simulink model "dab_fpga"  (R2024b)
settings: Solver=ode23tb  StartTime=0.0  StopTime=timeSpan  MaxStep=dab_maxstep  RelTol=1e-4
InitFcn:
  | p2s_dir = fileparts(get_param(bdroot, 'FileName'));
  | if ~isempty(p2s_dir), addpath(p2s_dir); end
  | clear p2s_dir
  | dab_params;
values from neighbouring files (symbols this model uses):
  AvergingTime = 1/(SwitchingFrequency/50)    (= 0.000333333333333)    [dab_params.m]
  dab_pid_avg_T = 1/(SwitchingFrequency*0.5)    (= 1.33333333333e-05)    [dab_params.m]
  DeadTime = 100e-9    (= 1e-07)    [dab_params.m]
  Dp = 1.0    (= 1)    [dab_params.m]
  Ds = 0.95    [dab_params.m]
  Force = 1    [dab_params.m]
  n_pri = 11    [dab_params.m]
  n_sec = 4    [dab_params.m]
  Pdab = struct()    [dab_params.m]
  Pout = 16000    [dab_params.m]
  SwitchingFrequency = 150e3    (= 150000)    [dab_params.m]
  tpsDpIntercept = 1.0    (= 1)    [dab_params.m]
  tpsDpMax = 1.0    (= 1)    [dab_params.m]
  tpsDpMin = 1.0    (= 1)    [dab_params.m]
  tpsDpSlope = 0.0    (= 0)    [dab_params.m]
  tpsDsIntercept = 0.95    [dab_params.m]
  tpsDsMax = 0.95    [dab_params.m]
  tpsDsMin = 0.95    [dab_params.m]
  tpsDsSlope = 0.0    (= 0)    [dab_params.m]
  Ts = 1/SwitchingFrequency    (= 6.66666666667e-06)    [dab_params.m]
  Vout = 250    [dab_params.m]
undefined symbols (not defined in the file or in its folder): dab_pid, dab_y0
libraries: slpidlib x1
Description:
  | Ideal-switch translation of DAB FPGA.plecs (see README.md)
settings Model: Creator=Jonathan  LastModifiedBy=Jonathan
settings SolverCC: ZeroCrossAlgorithm=Adaptive
settings DebuggingCC: MaxConsecutiveZCsMsg=none

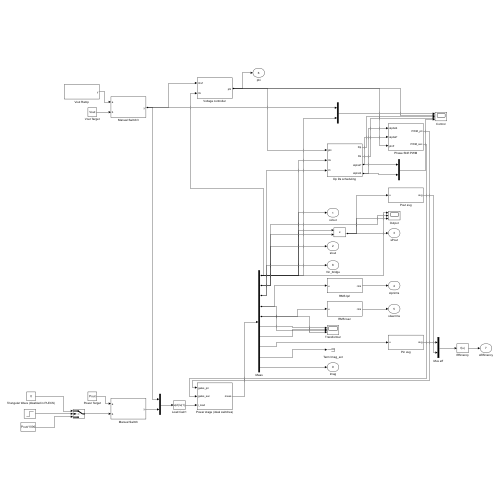
[thumbnail: Simulink's stored preview of the top-level diagram]
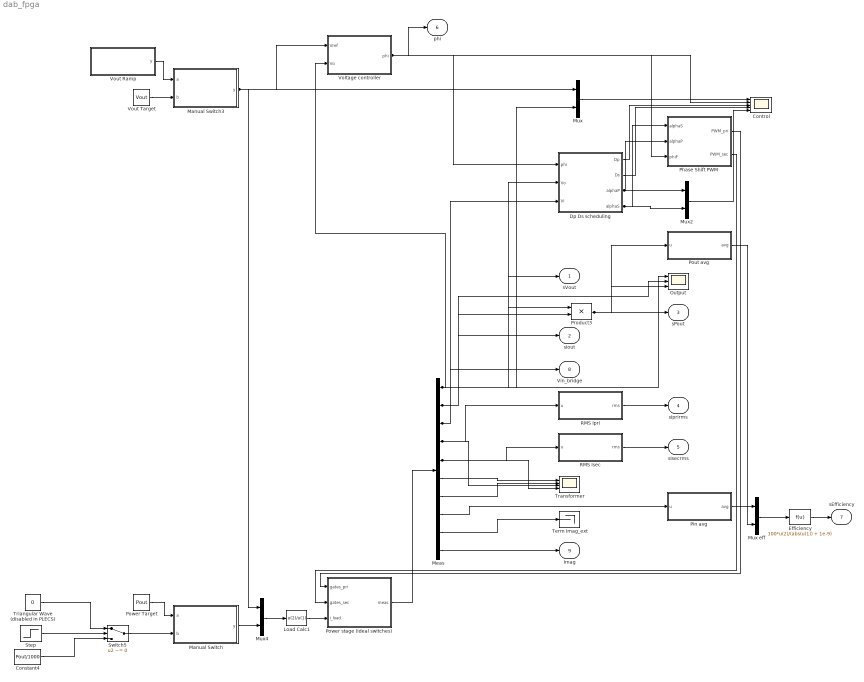
== system dab_fpga ==
  Constant4 : Constant  Value=Pout/1000
  Control : Scope  NumInputPorts=5
  Dp Ds scheduling : Subsystem
  Efficiency : Fcn  Expr=100*u(2)/(abs(u(1)) + 1e-9)
  Load Calc1 : Fcn  Expr=u(2)/u(1)
  Manual Switch : Subsystem
  Manual Switch3 : Subsystem
  Meas : Demux  Outputs=10
  Mux : Mux  Inputs=2
  Mux eff : Mux  Inputs=2
  Mux2 : Mux  Inputs=2
  Mux4 : Mux  Inputs=2
  Output : Scope  NumInputPorts=3
  Phase Shift PWM : Subsystem
  Pin avg : Subsystem
  Pout avg : Subsystem
  Power Target : Constant  Value=Pout
  Power stage (ideal switches) : Subsystem
  Product3 : Product  Inputs=**
  RMS Ipri : Subsystem
  RMS Isec : Subsystem
  Step : Step  Time=0.25  SampleTime=0
  Switch5 : Switch  Criteria=u2 ~= 0  SaturateOnIntegerOverflow=off  InputSameDT=off
  Term Imag_ext : Terminator
  Transformer : Scope  NumInputPorts=4
  Triangular Wave (disabled in PLECS) : Constant  Value=0
  Voltage controller : Subsystem
  Vout Ramp : Subsystem
  Vout Target : Constant  Value=Vout
  sVout : Outport
  sIout : Outport  Port=2
  sPout : Outport  Port=3
  sIprirms : Outport  Port=4
  sIsecrms : Outport  Port=5
  phi : Outport  Port=6
  sEfficiency : Outport  Port=7
  Vin_bridge : Outport  Port=8
  Imag : Outport  Port=9
  wires:
  Switch5/1 -> Manual Switch/2(b)
  Constant4/1 -> Switch5/3
  Power Target/1 -> Manual Switch/1(a)
  Step/1 -> Switch5/2
  Triangular Wave (disabled in PLECS)/1 -> Switch5/1
  Meas/7 -> Transformer/2
  Vout Ramp/1(y) -> Manual Switch3/1(a)
  Manual Switch3/1(y) -> Mux/1, Mux4/1, Voltage controller/1(Vref)
  Mux/1 -> Control/1
  Vout Target/1 -> Manual Switch3/2(b)
  RMS Ipri/1(rms) -> sIprirms/1
  Load Calc1/1 -> Power stage (ideal switches)/3(i_load)
  Manual Switch/1(y) -> Mux4/2
  Mux4/1 -> Load Calc1/1
  Voltage controller/1(phi) -> Control/2, Phase Shift PWM/3(phiF), Dp Ds scheduling/1(phi), phi/1
  Power stage (ideal switches)/1(meas) -> Meas/1
  Efficiency/1 -> sEfficiency/1
  Dp Ds scheduling/2(Ds) -> Control/4
  Meas/1 -> Voltage controller/2(Vo), Dp Ds scheduling/2(Vo), Product3/1, Output/1, sVout/1, Mux/2
  Meas/10 -> Imag/1
  Meas/2 -> Output/2, Product3/2, sIout/1
  Mux eff/1 -> Efficiency/1
  Meas/3 -> Vin_bridge/1, Dp Ds scheduling/3(Vi)
  Meas/4 -> RMS Ipri/1(u), Transformer/3
  Meas/5 -> RMS Isec/1(u), Transformer/4
  Mux2/1 -> Control/5
  Meas/6 -> Transformer/1
  Dp Ds scheduling/3(alphaP) -> Phase Shift PWM/2(alphaP), Mux2/1
  Meas/8 -> Pin avg/1(u)
  Product3/1 -> Pout avg/1(u), Output/3, sPout/1
  Meas/9 -> Term Imag_ext/1
  Dp Ds scheduling/1(Dp) -> Control/3
  Dp Ds scheduling/4(alphaS) -> Phase Shift PWM/1(alphaS), Mux2/2
  RMS Isec/1(rms) -> sIsecrms/1
  Phase Shift PWM/1(PWM_pri) -> Power stage (ideal switches)/1(gates_pri)
  Phase Shift PWM/2(PWM_sec) -> Power stage (ideal switches)/2(gates_sec)
  Pout avg/1(avg) -> Mux eff/2
  Pin avg/1(avg) -> Mux eff/1

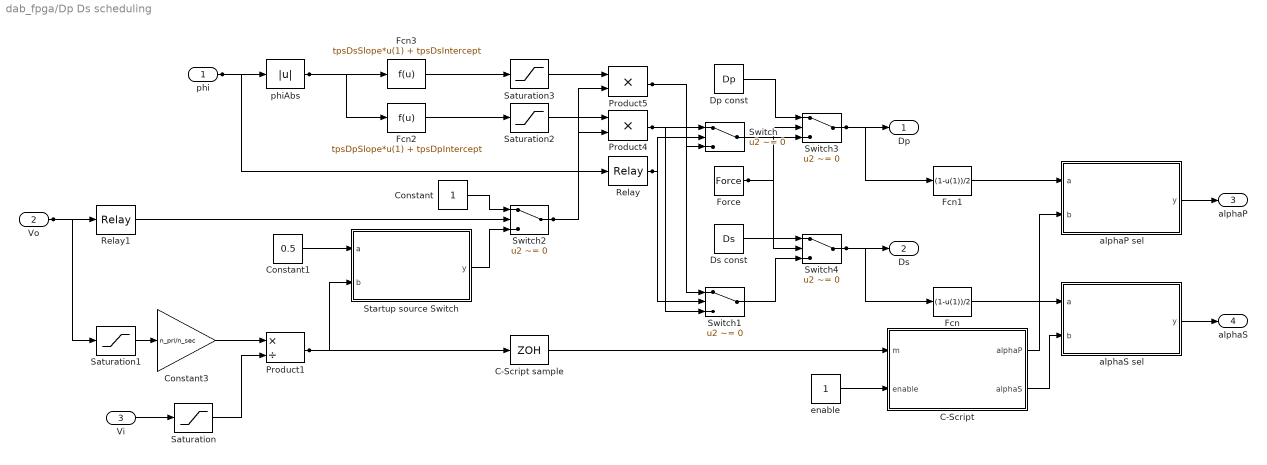
== system dab_fpga/Dp Ds scheduling ==
  phi : Inport
  Vo : Inport  Port=2
  Vi : Inport  Port=3
  C-Script : MATLAB Function  TreatAsAtomicUnit=on
  C-Script sample : ZeroOrderHold  SampleTime=Ts/10
  Constant : Constant
  Constant1 : Constant  Value=0.5
  Constant3 : Gain  Gain=n_pri/n_sec
  Dp const : Constant  Value=Dp
  Ds const : Constant  Value=Ds
  Fcn : Fcn  Expr=(1-u(1))/2
  Fcn1 : Fcn  Expr=(1-u(1))/2
  Fcn2 : Fcn  Expr=tpsDpSlope*u(1) + tpsDpIntercept
  Fcn3 : Fcn  Expr=tpsDsSlope*u(1) + tpsDsIntercept
  Force : Constant  Value=Force
  Product1 : Product  Inputs=*/
  Product4 : Product  Inputs=**
  Product5 : Product  Inputs=**
  Relay : Relay  OnSwitchValue=0.01  OffSwitchValue=-0.01
  Relay1 : Relay  OnSwitchValue=Vout  OffSwitchValue=Vout - 150
  Saturation : Saturate  UpperLimit=inf  LowerLimit=1
  Saturation1 : Saturate  UpperLimit=inf  LowerLimit=50
  Saturation2 : Saturate  UpperLimit=tpsDpMax  LowerLimit=tpsDpMin
  Saturation3 : Saturate  UpperLimit=tpsDsMax  LowerLimit=tpsDsMin
  Startup source Switch : Subsystem
  Switch{,1..4} (5 alike) : Switch  Criteria=u2 ~= 0  SaturateOnIntegerOverflow=off  InputSameDT=off
  alphaP sel : Subsystem
  alphaS sel : Subsystem
  enable : Constant
  phiAbs : Abs  SaturateOnIntegerOverflow=off
  Dp : Outport
  Ds : Outport  Port=2
  alphaP : Outport  Port=3
  alphaS : Outport  Port=4
  wires:
  Vo/1 -> Relay1/1, Saturation1/1
  Saturation1/1 -> Constant3/1
  Relay1/1 -> Switch2/2
  Vi/1 -> Saturation/1
  Saturation/1 -> Product1/2
  phi/1 -> Relay/1, phiAbs/1
  phiAbs/1 -> Fcn2/1, Fcn3/1
  Constant3/1 -> Product1/1
  Constant1/1 -> Startup source Switch/1(a)
  Product1/1 -> C-Script sample/1, Startup source Switch/2(b)
  Fcn3/1 -> Saturation3/1
  Fcn2/1 -> Saturation2/1
  Constant/1 -> Switch2/1
  Startup source Switch/1(y) -> Switch2/3
  Relay/1 -> Switch/2, Switch1/2
  Saturation3/1 -> Product5/1
  Saturation2/1 -> Product4/1
  Switch2/1 -> Product4/2, Product5/2
  C-Script sample/1 -> C-Script/1(m)
  Force/1 -> Switch3/2, Switch4/2
  Product5/1 -> Switch/3, Switch1/1
  Product4/1 -> Switch/1, Switch1/3
  Dp const/1 -> Switch3/1
  Switch/1 -> Switch3/3
  Ds const/1 -> Switch4/1
  Switch1/1 -> Switch4/3
  Switch3/1 -> Fcn1/1, Dp/1
  Switch4/1 -> Ds/1, Fcn/1
  enable/1 -> C-Script/2(enable)
  Fcn1/1 -> alphaP sel/1(a)
  Fcn/1 -> alphaS sel/1(a)
  C-Script/1(alphaP) -> alphaP sel/2(b)
  C-Script/2(alphaS) -> alphaS sel/2(b)
  alphaP sel/1(y) -> alphaP/1
  alphaS sel/1(y) -> alphaS/1

== system dab_fpga/Manual Switch ==
  a : Inport
  b : Inport  Port=2
  Switch : Switch  Criteria=u2 > Threshold  Threshold=0.5  SaturateOnIntegerOverflow=off  InputSameDT=off
  sel : Constant  Value=double(sel_power == 1)
  y : Outport
  wires:
  b/1 -> Switch/3
  a/1 -> Switch/1
  Switch/1 -> y/1
  sel/1 -> Switch/2

== system dab_fpga/Manual Switch3 ==
  a : Inport
  b : Inport  Port=2
  Switch : Switch  Criteria=u2 > Threshold  Threshold=0.5  SaturateOnIntegerOverflow=off  InputSameDT=off
  sel : Constant  Value=double(sel_vref == 1)
  y : Outport
  wires:
  Switch/1 -> y/1
  b/1 -> Switch/3
  sel/1 -> Switch/2
  a/1 -> Switch/1

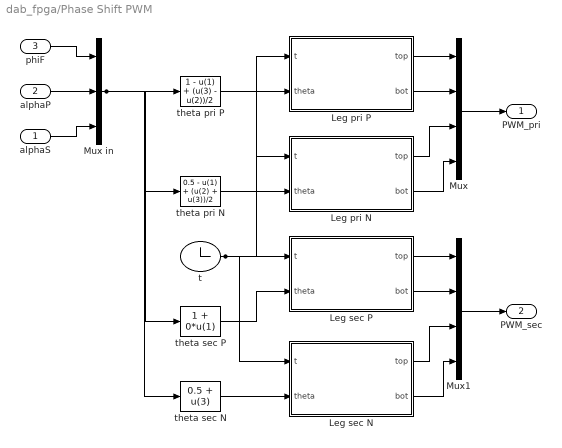
== system dab_fpga/Phase Shift PWM ==
  alphaS : Inport
  alphaP : Inport  Port=2
  phiF : Inport  Port=3
  Leg pri N : Subsystem
  Leg pri P : Subsystem
  Leg sec N : Subsystem
  Leg sec P : Subsystem
  Mux : Mux
  Mux in : Mux  Inputs=3
  Mux1 : Mux
  t : Clock
  theta pri N : Fcn  Expr=0.5 - u(1) + (u(2) + u(3))/2
  theta pri P : Fcn  Expr=1 - u(1) + (u(3) - u(2))/2
  theta sec N : Fcn  Expr=0.5 + u(3)
  theta sec P : Fcn  Expr=1 + 0*u(1)
  PWM_pri : Outport
  PWM_sec : Outport  Port=2
  wires:
  phiF/1 -> Mux in/1
  theta pri N/1 -> Leg pri N/2(theta)
  alphaP/1 -> Mux in/2
  theta sec P/1 -> Leg sec P/2(theta)
  alphaS/1 -> Mux in/3
  Mux in/1 -> theta pri P/1, theta pri N/1, theta sec P/1, theta sec N/1
  theta pri P/1 -> Leg pri P/2(theta)
  t/1 -> Leg pri P/1(t), Leg sec P/1(t), Leg pri N/1(t), Leg sec N/1(t)
  theta sec N/1 -> Leg sec N/2(theta)
  Leg pri P/1(top) -> Mux/1
  Leg pri P/2(bot) -> Mux/2
  Leg pri N/1(top) -> Mux/3
  Leg pri N/2(bot) -> Mux/4
  Leg sec P/1(top) -> Mux1/1
  Leg sec P/2(bot) -> Mux1/2
  Leg sec N/1(top) -> Mux1/3
  Leg sec N/2(bot) -> Mux1/4
  Mux/1 -> PWM_pri/1
  Mux1/1 -> PWM_sec/1

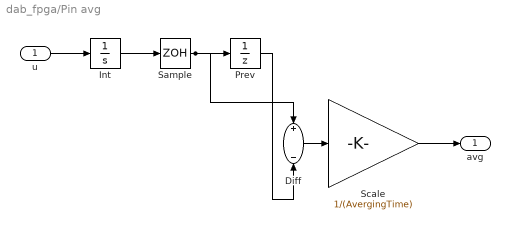
== system dab_fpga/Pin avg ==
  u : Inport
  Diff : Sum  Inputs=+-
  Int : Integrator
  Prev : UnitDelay  SampleTime=AvergingTime  HasFrameUpgradeWarning=on
  Sample : ZeroOrderHold  SampleTime=AvergingTime
  Scale : Gain  Gain=1/(AvergingTime)
  avg : Outport
  wires:
  u/1 -> Int/1
  Int/1 -> Sample/1
  Sample/1 -> Diff/1, Prev/1
  Prev/1 -> Diff/2
  Diff/1 -> Scale/1
  Scale/1 -> avg/1

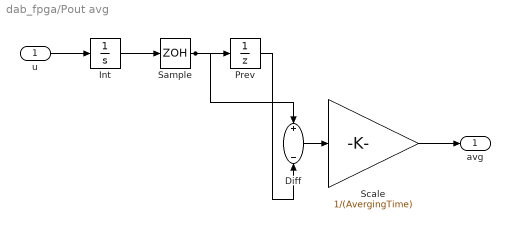
== system dab_fpga/Pout avg ==
  u : Inport
  Diff : Sum  Inputs=+-
  Int : Integrator
  Prev : UnitDelay  SampleTime=AvergingTime  HasFrameUpgradeWarning=on
  Sample : ZeroOrderHold  SampleTime=AvergingTime
  Scale : Gain  Gain=1/(AvergingTime)
  avg : Outport
  wires:
  Diff/1 -> Scale/1
  u/1 -> Int/1
  Int/1 -> Sample/1
  Sample/1 -> Diff/1, Prev/1
  Prev/1 -> Diff/2
  Scale/1 -> avg/1

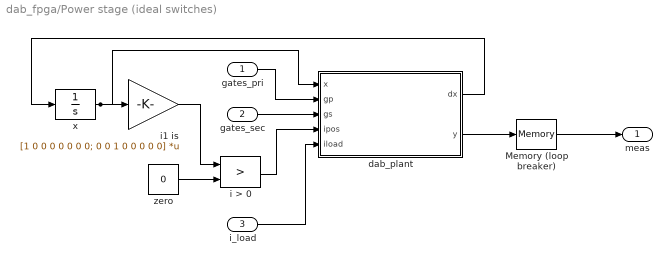
== system dab_fpga/Power stage (ideal switches) ==
  gates_pri : Inport
  gates_sec : Inport  Port=2
  i_load : Inport  Port=3
  Memory (loop breaker) : Memory  InitialCondition=dab_y0
  dab_plant : MATLAB Function  TreatAsAtomicUnit=on
  i > 0 : RelationalOperator  Operator=>  OutDataTypeStr=boolean  RndMeth=Simplest  InputSameDT=off
  i1 is : Gain  Gain=[1 0 0 0 0 0 0 0; 0 0 1 0 0 0 0 0]  Multiplication=Matrix(K*u)
  x : Integrator  InitialCondition=Pdab.x0
  zero : Constant  Value=0
  meas : Outport
  wires:
  i1 is/1 -> i > 0/1
  x/1 -> dab_plant/1(x), i1 is/1
  zero/1 -> i > 0/2
  gates_sec/1 -> dab_plant/3(gs)
  gates_pri/1 -> dab_plant/2(gp)
  i > 0/1 -> dab_plant/4(ipos)
  i_load/1 -> dab_plant/5(iload)
  dab_plant/1(dx) -> x/1
  dab_plant/2(y) -> Memory (loop breaker)/1
  Memory (loop breaker)/1 -> meas/1

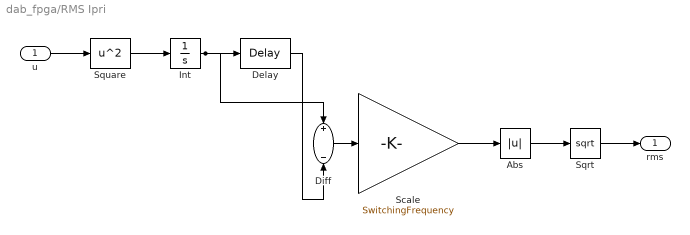
== system dab_fpga/RMS Ipri ==
  u : Inport
  Abs : Abs  SaturateOnIntegerOverflow=off
  Delay : TransportDelay  DelayTime=1/(SwitchingFrequency)  BufferSize=131072
  Diff : Sum  Inputs=+-
  Int : Integrator
  Scale : Gain  Gain=SwitchingFrequency
  Sqrt : Sqrt
  Square : Math  Operator=square
  rms : Outport
  wires:
  u/1 -> Square/1
  Scale/1 -> Abs/1
  Square/1 -> Int/1
  Abs/1 -> Sqrt/1
  Int/1 -> Diff/1, Delay/1
  Sqrt/1 -> rms/1
  Delay/1 -> Diff/2
  Diff/1 -> Scale/1

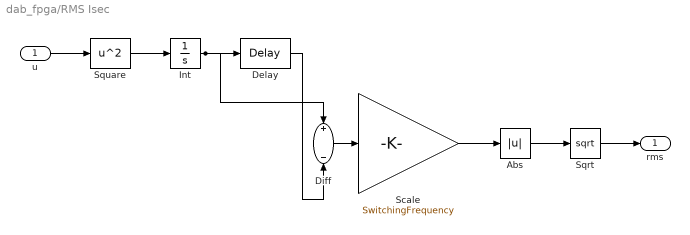
== system dab_fpga/RMS Isec ==
  u : Inport
  Abs : Abs  SaturateOnIntegerOverflow=off
  Delay : TransportDelay  DelayTime=1/(SwitchingFrequency)  BufferSize=131072
  Diff : Sum  Inputs=+-
  Int : Integrator
  Scale : Gain  Gain=SwitchingFrequency
  Sqrt : Sqrt
  Square : Math  Operator=square
  rms : Outport
  wires:
  Diff/1 -> Scale/1
  u/1 -> Square/1
  Abs/1 -> Sqrt/1
  Square/1 -> Int/1
  Sqrt/1 -> rms/1
  Int/1 -> Diff/1, Delay/1
  Delay/1 -> Diff/2
  Scale/1 -> Abs/1

== system dab_fpga/Voltage controller ==
  Vref : Inport
  Vo : Inport  Port=2
  Continuous PID Controller : slpidlib/PID Controller  Controller=PI  Form=Parallel  TimeDomain=Continuous-time  UseExternalTs=off  SampleTime=-1  IntegratorMethod=Forward Euler  FilterMethod=Forward Euler  ControllerParametersSource=internal  P=dab_pid.kp  I=dab_pid.ki  UseKiTs=off  D=0  UseExternalDerivativeSource=off  N=100  UseFilter=on  TunerSelectOption=Transfer Function Based (PID Tuner App)  InitialConditionSource=internal  InitialConditionForIntegrator=dab_pid.x0  InitialConditionForFilter=0  DifferentiatorICPrevScaledInput=0  ExternalReset=none  TrackingMode=off  Kt=1  LimitOutput=on  SatLimitsSource=internal  UpperSaturationLimit=dab_pid.up  LowerSaturationLimit=dab_pid.lo  LinearizeAsGain=on  AntiWindupMode=back-calculation  Kb=dab_pid.kbc  LimitIntegrator=off  UpperIntegratorSaturationLimit=inf  LowerIntegratorSaturationLimit=-inf  POutMin=[]  POutMax=[]  IOutMin=[]  IOutMax=[]  DOutMin=[]  DOutMax=[]  NOutMin=[]  NOutMax=[]  SumOutMin=[]  SumOutMax=[]  SaturationOutMin=[]  SaturationOutMax=[]  PParamMin=[]  PParamMax=[]  IParamMin=[]  IParamMax=[]  DParamMin=[]  DParamMax=[]  NParamMin=[]  NParamMax=[]  KbParamMin=[]  KbParamMax=[]  KtParamMin=[]  KtParamMax=[]  KbOutMin=[]  KbOutMax=[]  KtOutMin=[]  KtOutMax=[]  IntegratorOutMin=[]  IntegratorOutMax=[]  FilterOutMin=[]  FilterOutMax=[]  SumI1OutMin=[]  SumI1OutMax=[]  SumI2OutMin=[]  SumI2OutMax=[]  SumI3OutMin=[]  SumI3OutMax=[]  SumI4OutMin=[]  SumI4OutMax=[]  SumDOutMin=[]  SumDOutMax=[]  DifferentiatorOutMin=[]  DifferentiatorOutMax=[]  FilterDiffOutCoefMin=[]  FilterDiffOutCoefMax=[]  ReciprocalOutMin=[]  ReciprocalOutMax=[]  SumDenOutMin=[]  SumDenOutMax=[]  SumNumOutMin=[]  SumNumOutMax=[]  DivideOutMin=[]  DivideOutMax=[]  UdiffTsProdOutMin=[]  UdiffTsProdOutMax=[]  NTsProdOutMin=[]  NTsProdOutMax=[]  UintegralTsProdOutMin=[]  UintegralTsProdOutMax=[]  UngainTsProdOutMin=[]  UngainTsProdOutMax=[]  ClampingZeroOutDataTypeStr=Inherit: Inherit via back propagation  ClampingZeroOutMin=[]  ClampingZeroOutMax=[]  FilterDenConstantOutDataTypeStr=Inherit: Inherit via back propagation  FilterDenConstantOutMin=[]  FilterDenConstantOutMax=[]  PCopyOutDataTypeStr=Inherit: Inherit via back propagation  PCopyOutMin=[]  PCopyOutMax=[]  NCopyOutDataTypeStr=Inherit: Inherit via back propagation  NCopyOutMin=[]  NCopyOutMax=[]  IntegratorContinuousStateAttributes=''  IntegratorStateMustResolveToSignalObject=off  IntegratorRTWStateStorageClass=Auto  FilterContinuousStateAttributes=''  FilterStateMustResolveToSignalObject=off  FilterRTWStateStorageClass=Auto  ParallelPVariant=InternalParameters  IdealPVariant=Disabled  IVariant=InternalParameters  DVariant=Disabled  IntegratorVariant=Continuous  SatVariant=Enabled  AWVariant=BackCalculation  PCopyVariant=Disabled  TRVariant=Disabled  FdbkBlocksVariant=Forward  IdealPFdbkVariant=Disabled  SatFdbkVariant=Disabled  DerivativeFilterVariant=Disabled  NVariant=Disabled  NCopyVariant=Disabled_SignalSpec  FilterICVariant=Disabled  IntegratorICVariant=InternalICs  ExternalResetVariant=Disabled  TRSumVariant=Passthrough  SumFdbkVariant=Disabled  SumVariant=Sum_PI  TsampFilterVariant=InternalTs  TsampNgainVariant=Passthrough  TsampIntegralVariant=Disabled_SignalSpec  ExternalSaturationOutDataTypeStr=Inherit: Same as second input  DerivativeSourceVariant=Disabled  PreIntVariant=InternalPreInt
  Gain : Gain  Gain=0.5
  Periodic Average5 : Subsystem
  Sum2 : Sum  Inputs=+-
  phi : Outport
  wires:
  Vref/1 -> Sum2/1
  Gain/1 -> phi/1
  Periodic Average5/1(avg) -> Continuous PID Controller/1
  Sum2/1 -> Periodic Average5/1(u)
  Vo/1 -> Sum2/2
  Continuous PID Controller/1 -> Gain/1

== system dab_fpga/Vout Ramp ==
  Limit : Saturate  UpperLimit=max(0.1,Vout)  LowerLimit=min(0.1,Vout)
  Ramp : Fcn  Expr=(0.1) + (1600)*(u(1)-(0.0))*(u(1)>(0.0))
  t : Clock
  y : Outport
  wires:
  t/1 -> Ramp/1
  Ramp/1 -> Limit/1
  Limit/1 -> y/1

== system dab_fpga/Dp Ds scheduling/Startup source Switch ==
  a : Inport
  b : Inport  Port=2
  Switch : Switch  Criteria=u2 > Threshold  Threshold=0.5  SaturateOnIntegerOverflow=off  InputSameDT=off
  sel : Constant  Value=double(sel_startup == 1)
  y : Outport
  wires:
  a/1 -> Switch/1
  sel/1 -> Switch/2
  b/1 -> Switch/3
  Switch/1 -> y/1

== system dab_fpga/Dp Ds scheduling/alphaP sel ==
  a : Inport
  b : Inport  Port=2
  Switch : Switch  Criteria=u2 > Threshold  Threshold=0.5  SaturateOnIntegerOverflow=off  InputSameDT=off
  sel : Constant  Value=double(sel_alphaP == 1)
  y : Outport
  wires:
  a/1 -> Switch/1
  sel/1 -> Switch/2
  b/1 -> Switch/3
  Switch/1 -> y/1

== system dab_fpga/Dp Ds scheduling/alphaS sel ==
  a : Inport
  b : Inport  Port=2
  Switch : Switch  Criteria=u2 > Threshold  Threshold=0.5  SaturateOnIntegerOverflow=off  InputSameDT=off
  sel : Constant  Value=double(sel_alphaS == 1)
  y : Outport
  wires:
  a/1 -> Switch/1
  Switch/1 -> y/1
  sel/1 -> Switch/2
  b/1 -> Switch/3

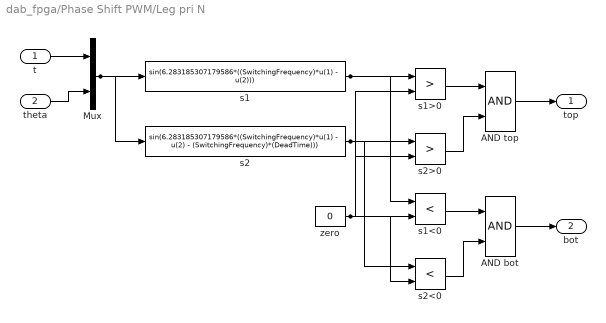
== system dab_fpga/Phase Shift PWM/Leg pri N ==
  t : Inport
  theta : Inport  Port=2
  AND bot : Logic  AllPortsSameDT=off  OutDataTypeStr=boolean
  AND top : Logic  AllPortsSameDT=off  OutDataTypeStr=boolean
  Mux : Mux  Inputs=2
  s1 : Fcn  Expr=sin(6.283185307179586*((SwitchingFrequency)*u(1) - u(2)))
  s1<0 : RelationalOperator  Operator=<  OutDataTypeStr=boolean  RndMeth=Simplest  InputSameDT=off
  s1>0 : RelationalOperator  Operator=>  OutDataTypeStr=boolean  RndMeth=Simplest  InputSameDT=off
  s2 : Fcn  Expr=sin(6.283185307179586*((SwitchingFrequency)*u(1) - u(2) - (SwitchingFrequency)*(DeadTime)))
  s2<0 : RelationalOperator  Operator=<  OutDataTypeStr=boolean  RndMeth=Simplest  InputSameDT=off
  s2>0 : RelationalOperator  Operator=>  OutDataTypeStr=boolean  RndMeth=Simplest  InputSameDT=off
  zero : Constant  Value=0
  top : Outport
  bot : Outport  Port=2
  wires:
  t/1 -> Mux/1
  theta/1 -> Mux/2
  s2>0/1 -> AND top/2
  zero/1 -> s2>0/2, s1>0/2, s1<0/2, s2<0/2
  Mux/1 -> s1/1, s2/1
  s1/1 -> s1>0/1, s1<0/1
  s2/1 -> s2>0/1, s2<0/1
  s1>0/1 -> AND top/1
  s1<0/1 -> AND bot/1
  s2<0/1 -> AND bot/2
  AND top/1 -> top/1
  AND bot/1 -> bot/1

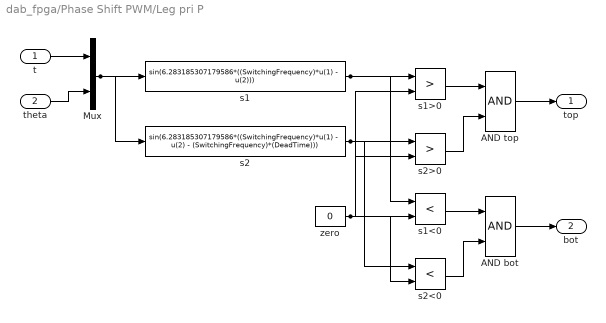
== system dab_fpga/Phase Shift PWM/Leg pri P ==
  t : Inport
  theta : Inport  Port=2
  AND bot : Logic  AllPortsSameDT=off  OutDataTypeStr=boolean
  AND top : Logic  AllPortsSameDT=off  OutDataTypeStr=boolean
  Mux : Mux  Inputs=2
  s1 : Fcn  Expr=sin(6.283185307179586*((SwitchingFrequency)*u(1) - u(2)))
  s1<0 : RelationalOperator  Operator=<  OutDataTypeStr=boolean  RndMeth=Simplest  InputSameDT=off
  s1>0 : RelationalOperator  Operator=>  OutDataTypeStr=boolean  RndMeth=Simplest  InputSameDT=off
  s2 : Fcn  Expr=sin(6.283185307179586*((SwitchingFrequency)*u(1) - u(2) - (SwitchingFrequency)*(DeadTime)))
  s2<0 : RelationalOperator  Operator=<  OutDataTypeStr=boolean  RndMeth=Simplest  InputSameDT=off
  s2>0 : RelationalOperator  Operator=>  OutDataTypeStr=boolean  RndMeth=Simplest  InputSameDT=off
  zero : Constant  Value=0
  top : Outport
  bot : Outport  Port=2
  wires:
  t/1 -> Mux/1
  theta/1 -> Mux/2
  s2>0/1 -> AND top/2
  zero/1 -> s2>0/2, s1<0/2, s1>0/2, s2<0/2
  Mux/1 -> s1/1, s2/1
  s1/1 -> s1>0/1, s1<0/1
  s2/1 -> s2>0/1, s2<0/1
  s1>0/1 -> AND top/1
  s1<0/1 -> AND bot/1
  s2<0/1 -> AND bot/2
  AND top/1 -> top/1
  AND bot/1 -> bot/1

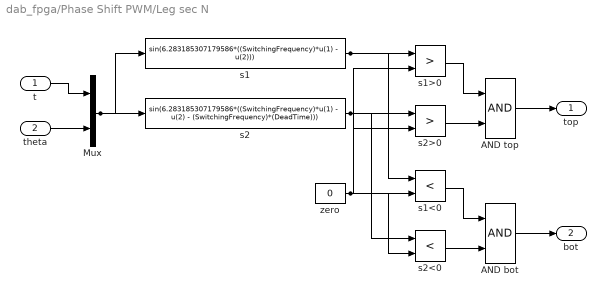
== system dab_fpga/Phase Shift PWM/Leg sec N ==
  t : Inport
  theta : Inport  Port=2
  AND bot : Logic  AllPortsSameDT=off  OutDataTypeStr=boolean
  AND top : Logic  AllPortsSameDT=off  OutDataTypeStr=boolean
  Mux : Mux  Inputs=2
  s1 : Fcn  Expr=sin(6.283185307179586*((SwitchingFrequency)*u(1) - u(2)))
  s1<0 : RelationalOperator  Operator=<  OutDataTypeStr=boolean  RndMeth=Simplest  InputSameDT=off
  s1>0 : RelationalOperator  Operator=>  OutDataTypeStr=boolean  RndMeth=Simplest  InputSameDT=off
  s2 : Fcn  Expr=sin(6.283185307179586*((SwitchingFrequency)*u(1) - u(2) - (SwitchingFrequency)*(DeadTime)))
  s2<0 : RelationalOperator  Operator=<  OutDataTypeStr=boolean  RndMeth=Simplest  InputSameDT=off
  s2>0 : RelationalOperator  Operator=>  OutDataTypeStr=boolean  RndMeth=Simplest  InputSameDT=off
  zero : Constant  Value=0
  top : Outport
  bot : Outport  Port=2
  wires:
  t/1 -> Mux/1
  s2/1 -> s2>0/1, s2<0/1
  theta/1 -> Mux/2
  s2>0/1 -> AND top/2
  Mux/1 -> s2/1, s1/1
  s1/1 -> s1>0/1, s1<0/1
  zero/1 -> s2>0/2, s1<0/2, s1>0/2, s2<0/2
  s1>0/1 -> AND top/1
  s1<0/1 -> AND bot/1
  s2<0/1 -> AND bot/2
  AND top/1 -> top/1
  AND bot/1 -> bot/1

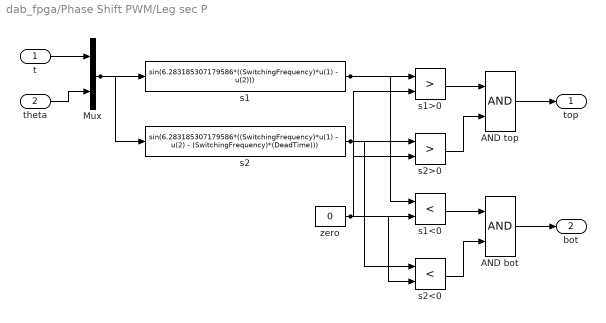
== system dab_fpga/Phase Shift PWM/Leg sec P ==
  t : Inport
  theta : Inport  Port=2
  AND bot : Logic  AllPortsSameDT=off  OutDataTypeStr=boolean
  AND top : Logic  AllPortsSameDT=off  OutDataTypeStr=boolean
  Mux : Mux  Inputs=2
  s1 : Fcn  Expr=sin(6.283185307179586*((SwitchingFrequency)*u(1) - u(2)))
  s1<0 : RelationalOperator  Operator=<  OutDataTypeStr=boolean  RndMeth=Simplest  InputSameDT=off
  s1>0 : RelationalOperator  Operator=>  OutDataTypeStr=boolean  RndMeth=Simplest  InputSameDT=off
  s2 : Fcn  Expr=sin(6.283185307179586*((SwitchingFrequency)*u(1) - u(2) - (SwitchingFrequency)*(DeadTime)))
  s2<0 : RelationalOperator  Operator=<  OutDataTypeStr=boolean  RndMeth=Simplest  InputSameDT=off
  s2>0 : RelationalOperator  Operator=>  OutDataTypeStr=boolean  RndMeth=Simplest  InputSameDT=off
  zero : Constant  Value=0
  top : Outport
  bot : Outport  Port=2
  wires:
  s1/1 -> s1>0/1, s1<0/1
  t/1 -> Mux/1
  theta/1 -> Mux/2
  s2>0/1 -> AND top/2
  Mux/1 -> s1/1, s2/1
  s2/1 -> s2>0/1, s2<0/1
  zero/1 -> s1<0/2, s1>0/2, s2<0/2, s2>0/2
  s1>0/1 -> AND top/1
  s1<0/1 -> AND bot/1
  s2<0/1 -> AND bot/2
  AND top/1 -> top/1
  AND bot/1 -> bot/1

== system dab_fpga/Voltage controller/Periodic Average5 ==
  u : Inport
  Diff : Sum  Inputs=+-
  Int : Integrator
  Prev : UnitDelay  SampleTime=dab_pid_avg_T  HasFrameUpgradeWarning=on
  Sample : ZeroOrderHold  SampleTime=dab_pid_avg_T
  Scale : Gain  Gain=1/(dab_pid_avg_T)
  avg : Outport
  wires:
  Sample/1 -> Prev/1, Diff/1
  Int/1 -> Sample/1
  u/1 -> Int/1
  Scale/1 -> avg/1
  Diff/1 -> Scale/1
  Prev/1 -> Diff/2

== matlab function dab_fpga/Dp Ds scheduling/C-Script ==
  data: m input; alphaP output; enable input; alphaS output
function [alphaP, alphaS] = dab_alpha_cscript(m, enable)
%DAB_ALPHA_CSCRIPT  Translation of the PLECS "C-Script" block in DAB FPGA.plecs: inner phase
%   shifts from the voltage gain m = Vo*n/Vi (minimum 0.045), zero when not enabled.
%#codegen
alphaP = 0;
alphaS = 0;
if enable == 1
    if m <= 1
        alphaP = max(0.5*(1 - m), 0.045);
        alphaS = 0.045;
    else
        alphaP = 0.045;
        alphaS = max(0.5*(1 - 1/m), 0.045);
    end
end
end

== matlab function dab_fpga/Power stage (ideal switches)/dab_plant ==
  data: dx output; x input size=[8 1]; y output; gp input size=[4 1]; gs input size=[4 1]; ipos input size=[2 1]; iload input size=1; Pdab parameter
function [dx, y] = dab_plant(x, gp, gs, ipos, iload, Pdab)
%DAB_PLANT  Ideal-switch power stage of "DAB FPGA.plecs" (body of the MATLAB Function block).
%
% Circuit (as in the PLECS schematic, primary bridge config "Infineon IMZC120R012M2H",
% secondary "Infineon IMZA65R007M2H", transformer config "Electrical"):
%
%   V_dc --R1--+-- DC+  [primary full bridge]  P --Llk(Llkp)--A--+--------------------+
%   (Vin)      |                                                  |                    |
%            Rcin                                          Llk1 (1.3 mH)   R5,Lp(Llk) --+ Tr2 (np:ns, Lm)
%            Cin                                                  |        R2 ---------+
%              |                                    N --Crp-------B--+--------------------+
%   ------- DC- ...
%   Tr2 secondary --Ls(Llk),R3--port3--Asec--Llk2(Llks)-- P [secondary full bridge] DC+ --+-- Co+R_Cout
%   Tr2 secondary --R4--port4--Crs-------------------- N                              +-- Cdc+R_Cdc
%                                                                                     +-- load current
%
% The MOSFETs are ideal switches with ideal anti-parallel diodes: a leg whose gates are both
% off (dead time) is clamped by the diode selected by the sign of its current. Snubbers
% (Csnub/Rsnub), Coss, the 55 pF inter-winding capacitance and the thermal/loss network are
% not modelled (switching dynamics only).
%
% States  x = [i1; ip; is; vCrp; vCrs; vCin; vCo; vCdc]
%   i1   current in the external primary leakage Llk (out of primary bridge P terminal)
%   ip   current in the transformer-internal primary leakage Lp (into Tr2 dot)
%   is   secondary current (out of Tr2 secondary dot, into secondary bridge P terminal)
%   vCrp primary series capacitor voltage, vCrs secondary series capacitor voltage
%   vCin input capacitor, vCo / vCdc the two output capacitors (each behind its ESR)
% Inputs
%   gp    4 gate signals primary  [Q1 (P top) Q2 (P bottom) Q3 (N top) Q4 (N bottom)]
%   gs    4 gate signals secondary, same order
%   ipos  [i1 > 0; is > 0]  (computed outside from the states so that the solver gets a
%         zero-crossing event when a diode current reverses)
%   iload load current drawn from the output node (A)
% Outputs
%   dx  state derivatives
%   y   [Vo; Io; Vin_bridge; i1; is; v_pri_bridge; v_sec_bridge; Pin; i_mag_ext; i_mag]
%#codegen

P = Pdab;   % parameter struct from the workspace

i1 = x(1); ip = x(2); is = x(3);
vCrp = x(4); vCrs = x(5); vCin = x(6); vCo = x(7); vCdc = x(8);

g1 = double(gp);
g2 = double(gs);
ip1 = double(ipos(1)) > 0.5;   % i1 > 0
is1 = double(ipos(2)) > 0.5;   % is > 0

% Leg output state: 1 = midpoint tied to DC+, 0 = tied to DC-.
% The current out of each leg midpoint is: pri P: +i1, pri N: -i1, sec P: -is, sec N: +is.
uPp = leg_state(g1(1), g1(2), ip1);
uNp = leg_state(g1(3), g1(4), ~ip1);
uPs = leg_state(g2(1), g2(2), ~is1);
uNs = leg_state(g2(3), g2(4), is1);

kp = uPp - uNp;          % primary bridge: v_ac = kp * v_dc, i_dc = kp * i_ac
ks = uPs - uNs;          % secondary bridge

% Primary DC node: source Vin behind R1 in parallel with Cin behind R_Cin
idcp = kp * i1;
vin = (P.Vin / P.R1 + vCin / P.RCin - idcp) / (1 / P.R1 + 1 / P.RCin);
vpb = kp * vin;

% Secondary DC node: Co behind R_Cout and Cdc behind R_Cdc in parallel, load current out
idcs = ks * is;
vo = (idcs - iload + vCo / P.RCo + vCdc / P.RCdc) / (1 / P.RCo + 1 / P.RCdc);
vsb = ks * vo;

% Coupled inductor equations M * d[i1; ip; is]/dt = rhs (M is constant, inverse precomputed)
rhs = [vpb - vCrp; -P.Rp * ip; -(P.Rs * is + vsb + vCrs)];
di = P.Minv * rhs;

dx = zeros(8, 1);
dx(1:3) = di;
dx(4) = i1 / P.Crp;
dx(5) = is / P.Crs;
dx(6) = (vin - vCin) / (P.RCin * P.Cin);
dx(7) = (vo - vCo) / (P.RCo * P.Co);
dx(8) = (vo - vCdc) / (P.RCdc * P.Cdc);

io = (vo - vCdc) / P.RCdc + iload;      % ammeter "Io" (into Cdc branch + load)
pin = P.Vin * (P.Vin - vin) / P.R1;     % power delivered by the DC source
y = [vo; io; vin; i1; is; vpb; vsb; pin; i1 - ip; ip - P.n * is];
end

function u = leg_state(top, bot, iout_pos)
% Ideal half bridge: gate wins, otherwise the anti-parallel diode picked by current direction
% (current flowing out of the midpoint is supplied by the bottom diode).
if top > 0.5
    u = 1;
elseif bot > 0.5
    u = 0;
elseif iout_pos
    u = 0;
else
    u = 1;
end
end
